simulink model "amdtector"  (R2022b)
settings: Solver=VariableStepAuto  StartTime=0.0  StopTime=0.1  RelTol=1e-3
undefined symbols (not defined in the file or in its folder): sigbuilder_block
libraries: fl_lib x11, nesl_utility x5, ee_lib x1
settings Model: Creator=fuad  LastModifiedBy=fuad

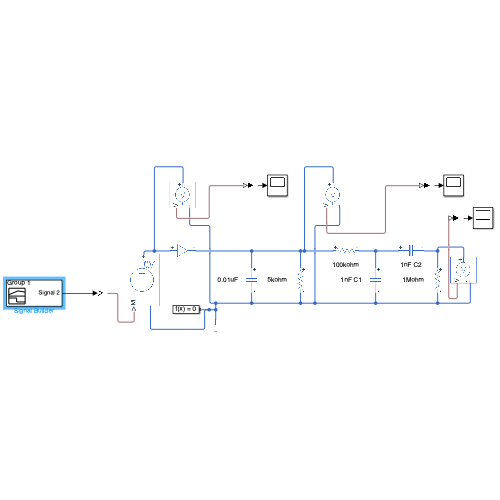
[thumbnail: Simulink's stored preview of the top-level diagram]
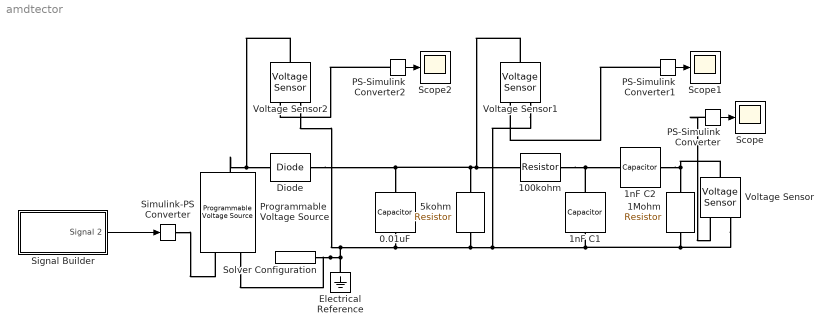
== system amdtector ==
  0.01uF : fl_lib/Electrical/Electrical Elements/Capacitor  c=0.01e-6 F  r=1e-6 Ohm  g=0 1/Ohm  i_specify=off  i_priority=None  i=0 A  i_nominal_specify=off  i_nominal_unit=A  i_nominal_value=1  v_specify=off  v_priority=None  v=0 V  v_nominal_specify=off  v_nominal_unit=V  v_nominal_value=1  vc_specify=off  vc_priority=High  vc=0 V  vc_nominal_specify=off  vc_nominal_unit=V  vc_nominal_value=1
  100kohm : fl_lib/Electrical/Electrical Elements/Resistor  R=100 kOhm  i_specify=off  i_priority=None  i=0 A  i_nominal_specify=off  i_nominal_unit=A  i_nominal_value=1  v_specify=off  v_priority=None  v=0 V  v_nominal_specify=off  v_nominal_unit=V  v_nominal_value=1
  1Mohm : fl_lib/Electrical/Electrical Elements/Resistor  R=1 MOhm  i_specify=off  i_priority=None  i=0 A  i_nominal_specify=off  i_nominal_unit=A  i_nominal_value=1  v_specify=off  v_priority=None  v=0 V  v_nominal_specify=off  v_nominal_unit=V  v_nominal_value=1
  1nF C1 : fl_lib/Electrical/Electrical Elements/Capacitor  c=1e-9 F  r=1e-6 Ohm  g=0 1/Ohm  i_specify=off  i_priority=None  i=0 A  i_nominal_specify=off  i_nominal_unit=A  i_nominal_value=1  v_specify=off  v_priority=None  v=0 V  v_nominal_specify=off  v_nominal_unit=V  v_nominal_value=1  vc_specify=off  vc_priority=High  vc=0 V  vc_nominal_specify=off  vc_nominal_unit=V  vc_nominal_value=1
  1nF C2 : fl_lib/Electrical/Electrical Elements/Capacitor  c=1e-9 F  r=1e-6 Ohm  g=0 1/Ohm  i_specify=off  i_priority=None  i=0 A  i_nominal_specify=off  i_nominal_unit=A  i_nominal_value=1  v_specify=off  v_priority=None  v=0 V  v_nominal_specify=off  v_nominal_unit=V  v_nominal_value=1  vc_specify=off  vc_priority=High  vc=0 V  vc_nominal_specify=off  vc_nominal_unit=V  vc_nominal_value=1
  5kohm : fl_lib/Electrical/Electrical Elements/Resistor  R=5 kOhm  i_specify=off  i_priority=None  i=0 A  i_nominal_specify=off  i_nominal_unit=A  i_nominal_value=1  v_specify=off  v_priority=None  v=0 V  v_nominal_specify=off  v_nominal_unit=V  v_nominal_value=1
  Diode : fl_lib/Electrical/Electrical Elements/Diode  Vf=0.6 V  Ron=0.3 Ohm  Goff=1e-8 1/Ohm  i_specify=off  i_priority=None  i=0 A  i_nominal_specify=off  i_nominal_unit=A  i_nominal_value=1  v_specify=off  v_priority=None  v=0 V  v_nominal_specify=off  v_nominal_unit=V  v_nominal_value=1
  Electrical Reference : fl_lib/Electrical/Electrical Elements/Electrical Reference
  PS-Simulink Converter : nesl_utility/PS-Simulink Converter  PhysicalDomain=network_engine_domain  SubClassName=ps_output  LeftPortType=input  RightPortType=output  PseudoPeriodic=off  Frequencies=[]  VectorFormat=inherit  Unit=inherit  AffineConversion=off
  PS-Simulink Converter1 : nesl_utility/PS-Simulink Converter  PhysicalDomain=network_engine_domain  SubClassName=ps_output  LeftPortType=input  RightPortType=output  PseudoPeriodic=off  Frequencies=[]  VectorFormat=inherit  Unit=inherit  AffineConversion=off
  PS-Simulink Converter2 : nesl_utility/PS-Simulink Converter  PhysicalDomain=network_engine_domain  SubClassName=ps_output  LeftPortType=input  RightPortType=output  PseudoPeriodic=off  Frequencies=[]  VectorFormat=inherit  Unit=inherit  AffineConversion=off
  Programmable Voltage Source : ee_lib/Sources/Programmable Voltage Source  magnitude_type=ee.enum.timechanging.external  ac_magnitude=100 V  magn_ramp=1 V/s  magn_step=1 V  magn_modu_magn=1 V  magn_modu_freq=1 Hz  magn_t1=1 s  magn_t2=2 s  frequency_type=ee.enum.timechanging.constant  ac_frequency=60 Hz  freq_ramp=1 Hz/s  freq_step=1 Hz  freq_modu_magn=1 Hz  freq_modu_freq=1 Hz  freq_t1=1 s  freq_t2=2 s  phase_type=ee.enum.timechanging.constant  ac_shift=0 deg  phase_ramp=1 deg/s  phase_step=1 deg  phase_modu_magn=1 deg  phase_modu_freq=1 Hz  phase_t1=1 s  phase_t2=2 s  dc_type=ee.enum.timechanging.constant  dc_voltage=0 V  dc_ramp=1 V/s  dc_step=1 V  dc_modu_magn=1 V  dc_modu_freq=1 Hz  dc_t1=1 s  dc_t2=2 s  harmonic_option=0  harmonic_orders=[5, 7, 11, 13]  harmonic_ratios=[.1, .1, .1, .1]  harmonic_shifts=[0, 0, 0, 0] deg  harmonic_t1=-inf s  harmonic_t2=inf s  noise_mode=0  PSD=0 V^2/Hz  repeatability=1  auto_seed=0  user_seed=0  sample_time=1e-3 s  i_specify=off  i_priority=None  i=0 A  i_nominal_specify=off  i_nominal_unit=A  i_nominal_value=1  v_specify=off  v_priority=None  v=0 V  v_nominal_specify=off  v_nominal_unit=V  v_nominal_value=1
      settings: InternalSimscapePortConfiguration="{\"Bottom\":[],\"Left\":[{\"id\":\"p\",\"label\":\"+\",\"type\":\"foundation.electrical.electrical\"}],\"Right\":[{\"id\":\"ext_magn\",\"label\":\"M\",\"type\":\"input\"},{\"id\":\"n\",\"label\":\"-\",\"type\":\"foundation.electrical.electrical\"}],\"Top\":[]}"
  Scope : Scope
  Scope1 : Scope
  Scope2 : Scope
  Signal Builder : Subsystem  Tag=STV Subsys  LoadFcn=sigbuilder_block('load');  StartFcn=sigbuilder_block('start');  StopFcn=sigbuilder_block('stop');  ClipboardFcn=sigbuilder_block('clipboard');  mask(Sigbuilder block){tuvar=[0:10]}
      mask help: Simulink:masks:SigbuilderBlock_MD
      mask init:
      | if ~strcmp(get_param(bdroot(gcbh),'SimulationStatus'),'stopped') tuvar = sigbuilder_block('maskInit'); end
      settings: CopyFcn=sigbuilder_block('copy');  DeleteFcn=sigbuilder_block('delete');  ModelCloseFcn=sigbuilder_block('modelClose');  PreSaveFcn=sigbuilder_block('preSave');  PauseFcn=sigbuilder_block('pause');  ContinueFcn=sigbuilder_block('continue');  NameChangeFcn=sigbuilder_block('namechange');  OpenFcn=sigbuilder_block('open',[0 51 1440 715 ]);  CloseFcn=sigbuilder_block('close');
      mask Display: plot(0, 0, 100, 100,[2, 2, 32, 32, 2], [68, 8, 8, 68, 68],[32, 2], [38, 38], [32, 19, 2],[53, 60, 44], [32, 17, 17, 2],[16, 16, 31, 31]);txt = getActiveGroup(gcbh);text(2, 100, txt,'verticalAlignment', 'top');
  Simulink-PS Converter : nesl_utility/Simulink-PS Converter  PhysicalDomain=network_engine_domain  SubClassName=ps_input  LeftPortType=input  RightPortType=output  PseudoPeriodic=off  Frequencies=[]  NoiseDistribution=none  NoiseParameters=[]  Unit=1  AffineConversion=off  FilteringAndDerivatives=provide  SimscapeFilterOrder=1  InputFilterTimeConstant=0.001  UdotUserProvided=0
  Solver Configuration : nesl_utility/Solver Configuration  PhysicalDomain=network_engine_domain  SubClassName=solver  LeftPortType=input  RightPortType=generic  Tones=[]  Harmonics=[]  SimulateNoise=off  Profile=off  UseLocalSampling=off  EnableSwitchedLinearOptims=on  FrequencyDomain=off  UseCCode=off  RelTol=0.001  AbsTol=0.001  MinStep=1e-09  ToWorkspace=off  RevertToSquareIcSolve=off  NumHomotopyIterations=100  PhasorMode=off  PhasorModeNumHarmonics=1  ConsistencySolver=NEWTON_XTOL_AFTER_FTOL  IndexReductionMethod=DerivativeReplacement  DoDC=off  ResidualTolerance=1e-09  ConsistencyTolSource=GLOBAL  ConsistencyAbsTol=0.001  ConsistencyRelTol=0.001  ConsistencyTolFactor=0.001  UseLocalSolver=off  LocalSolverChoice=NE_BACKWARD_EULER_ADVANCER  ResolveIndetEquations=on  FunctionEvalNumThread=1  LocalSolverSampleTime=0.001  DoFixedCost=off  MaxNonlinIter=3  MaxModeIter=2  ComputeImpulses=off  ImpulseIterations=2  LinearAlgebra=auto  LinearAlgebraNumThread=0  EquationFormulation=NE_TIME_EF  DelaysMemoryBudget=1024  AutomaticFiltering=on  FilteringTimeConstant=0.001  PartitionStorageMethod=AS_NEEDED  PartitionMemoryBudget=1024  PartitionMethod=ROBUST
  Voltage Sensor : fl_lib/Electrical/Electrical Sensors/Voltage Sensor
  Voltage Sensor1 : fl_lib/Electrical/Electrical Sensors/Voltage Sensor
  Voltage Sensor2 : fl_lib/Electrical/Electrical Sensors/Voltage Sensor
  wires:
  Signal Builder/1(Signal 2) -> Simulink-PS Converter/1
  PS-Simulink Converter/1 -> Scope/1
  PS-Simulink Converter1/1 -> Scope1/1
  PS-Simulink Converter2/1 -> Scope2/1
  connections:
  Voltage Sensor1/LConn1 -- 100kohm/LConn1 -- 5kohm/LConn1 -- Diode/RConn1 -- 0.01uF/LConn1
  100kohm/RConn1 -- 1nF C1/LConn1 -- 1nF C2/LConn1
  1nF C2/RConn1 -- Voltage Sensor/LConn1 -- 1Mohm/LConn1
  1Mohm/RConn1 -- Voltage Sensor/RConn2 -- Voltage Sensor2/RConn2 -- Programmable Voltage Source/RConn2 -- Solver Configuration/RConn1 -- Electrical Reference/LConn1 -- 0.01uF/RConn1 -- 5kohm/RConn1 -- Voltage Sensor1/RConn2 -- 1nF C1/RConn1
  Programmable Voltage Source/LConn1 -- Voltage Sensor2/LConn1 -- Diode/LConn1
  Simulink-PS Converter/RConn1 -- Programmable Voltage Source/RConn1
  PS-Simulink Converter/LConn1 -- Voltage Sensor/RConn1
  PS-Simulink Converter1/LConn1 -- Voltage Sensor1/RConn1
  PS-Simulink Converter2/LConn1 -- Voltage Sensor2/RConn1

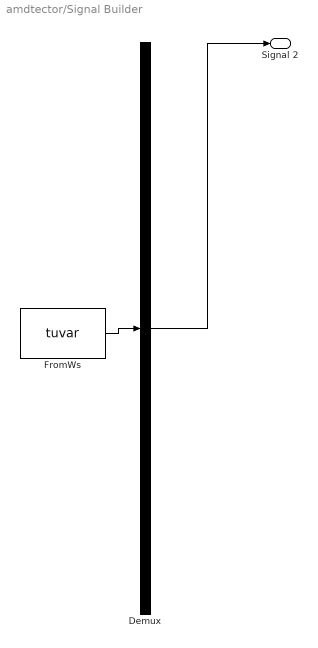
== system amdtector/Signal Builder ==
  Demux : Demux  Tag=STV Demux  Outputs=1
      settings: DisplayOption=none
  FromWs : FromWorkspace  Tag=STV FromWs  VariableName=tuvar
      SigBuilderData=|
      | common.afterFinalStr = 'Extrapolate'
      | common.sampleTime = 0
      | dataSet.timeRange = [0 10]
      | dataSet.name = 'Group 1'
      | sbobj.Groups.Name = 'Group 1'
      | sbobj.Groups.Signals.Name = 'Signal 2'
      | sbobj.Groups.Signals.XData = [0 9.99999999962e-06 1.99999999992e-05 2.99999999989e-05 3.99999999985e-05 4.99999999999e-05 5.99999999995e-05 6.99999999991e-05 7.99999999987e-05 8.99999999984e-05 9.99999999998e-05 0.000109999999999 ... (1000001 elements, 1x1000001)]
      | sbobj.Groups.Signals.YData = [180.000050171 179.641314986 178.566595733 176.780344928 174.289962155 171.10576225 167.240930955 162.711468248 157.536119591 151.736295411 145.335979162 138.361624396 ... (1000001 elements, 1x1000001)]
  Signal 2 : Outport  Tag=STV Outport
  wires:
  FromWs/1 -> Demux/1
  Demux/1 -> Signal 2/1
